simulink model "nmm2d"  (R2025a)
settings: Solver=ode15s  StartTime=0.0  StopTime=20  FixedStep=1e-3  MaxStep=ts_max  RelTol=1e-3  AbsTol=1e-4  EnableMultiTasking=on
values from neighbouring files (symbols this model uses):
  c = 0.05    [nmm2d_mInit.m]
  c_jointstop = 0.3 / (pi/180)    (= 17.1887338539)    [nmm2d_mInit.m]
  D12_F = 0.16    [nmm2d_mInit.m]
  D12_S = L_S    (= 0.5)    [nmm2d_mInit.m]
  D12_T = L_T    (= 0.5)    [nmm2d_mInit.m]
  D1G_F = 0.14    [nmm2d_mInit.m]
  D1G_HAT = 0.35    [nmm2d_mInit.m]
  D1G_S = 0.3    [nmm2d_mInit.m]
  D1G_T = 0.3    [nmm2d_mInit.m]
  DeltaThRef = 5e-3    (= 0.005)    [nmm2d_mInit.m]
  eref = 0.04    [nmm2d_mInit.m]
  FmaxVec = [FmaxSOL FmaxTA FmaxGAS FmaxVAS FmaxHAM FmaxGLU FmaxHFL               FmaxSOL FmaxTA FmaxGAS FmaxVAS FmaxHAM FmaxGLU FmaxHFL]'    [nmm2d_mInit.m]
  g = 9.81    [nmm2d_mInit.m]
  GainDeltaTheta = 2 /100*180/pi    (= 1.14591559026)    [nmm2d_cInit.m]
  GainGAS = 1.1/FmaxGAS    [nmm2d_cInit.m]
  GainGLU = 0.5/FmaxGLU    [nmm2d_cInit.m]
  GainHAM = 0.65/FmaxHAM    [nmm2d_cInit.m]
  GainHAMHFL = 4    [nmm2d_cInit.m]
  GainHFL = 0.5    [nmm2d_cInit.m]
  GainKneOverExt = 2    [nmm2d_cInit.m]
  GainSOL = 1.2/FmaxSOL    [nmm2d_cInit.m]
  GainSOLTA = 0.4/FmaxSOL    [nmm2d_cInit.m]
  GainTA = 1.1    [nmm2d_cInit.m]
  GainVAS = 1.2/FmaxVAS    [nmm2d_cInit.m]
  HAT_CG0 = [-D12_F; 0] + Rot120*[L_S;0] + Rot120*Rot230*[-L_T;0]            + Rot120*Rot230*Rot340*[D1G_HAT;0]    [nmm2d_cInit.m]
  In_F = 0.005    [nmm2d_mInit.m]
  In_HAT = 3    [nmm2d_mInit.m]
  In_S = 0.05    [nmm2d_mInit.m]
  In_T = 0.15    [nmm2d_mInit.m]
  K = 5    [nmm2d_mInit.m]
  k_gx = (2*(m_F+m_S+m_T)+m_HAT)*g/0.1    (= 7848)    [nmm2d_mInit.m]
  k_gy = (2*(m_F+m_S+m_T)+m_HAT)*g/0.01    (= 78480)    [nmm2d_mInit.m]
  k_pressure = m_HAT * 9.81 / DeltaThRef    (= 104967)    [nmm2d_mInit.m]
  K_swing = 0.25    [nmm2d_cInit.m]
  KneePh23Offset = 170*pi/180    (= 2.96705972839)    [nmm2d_cInit.m]
  L_F = 0.2    [nmm2d_mInit.m]
  L_HAT = 0.8    [nmm2d_mInit.m]
  L_S = 0.5    [nmm2d_mInit.m]
  L_T = 0.5    [nmm2d_mInit.m]
  LceOffsetHAM = 0.85    [nmm2d_cInit.m]
  LceOffsetHFL = 0.65    [nmm2d_cInit.m]
  LceOffsetTA = 1-0.5*w    [nmm2d_cInit.m]
  LongDelay = 0.020    (= 0.02)    [nmm2d_cInit.m]
  loptGAS = 0.05    [nmm2d_mInit.m]
  loptGLU = 0.11    [nmm2d_mInit.m]
  loptHAM = 0.10    (= 0.1)    [nmm2d_mInit.m]
  loptHFL = 0.11    [nmm2d_mInit.m]
  loptSOL = 0.04    [nmm2d_mInit.m]
  loptTA = 0.06    [nmm2d_mInit.m]
  loptVAS = 0.08    [nmm2d_mInit.m]
  loptVec = [loptSOL loptTA loptGAS loptVAS loptHAM loptGLU loptHFL               loptSOL loptTA loptGAS loptVAS loptHAM loptGLU loptHFL]'    [nmm2d_mInit.m]
  Lphi120 = 85*pi/180    (= 1.4835298642)    [nmm2d_cInit.m]
  Lphi230 = 175*pi/180    (= 3.05432619099)    [nmm2d_cInit.m]
  Lphi340 = 175*pi/180    (= 3.05432619099)    [nmm2d_cInit.m]
  lslackGAS = 0.40    (= 0.4)    [nmm2d_mInit.m]
  lslackGLU = 0.13    [nmm2d_mInit.m]
  lslackHAM = 0.31    [nmm2d_mInit.m]
  lslackHFL = 0.10    (= 0.1)    [nmm2d_mInit.m]
  lslackSOL = 0.26    [nmm2d_mInit.m]
  lslackTA = 0.24    [nmm2d_mInit.m]
  lslackVAS = 0.23    [nmm2d_mInit.m]
  lslackVec = [lslackSOL lslackTA lslackGAS lslackVAS lslackHAM lslackGLU lslackHFL                 lslackSOL lslackTA lslackGAS lslackVAS lslackHAM lslackGLU lslackHFL]'    [nmm2d_mInit.m]
  m_F = 1.25    [nmm2d_mInit.m]
  m_HAT = 53.5    [nmm2d_mInit.m]
  m_S = 3.5    [nmm2d_mInit.m]
  m_T = 8.5    [nmm2d_mInit.m]
  MidDelay = 0.010    (= 0.01)    [nmm2d_cInit.m]
  mu_slide = 0.8    [nmm2d_mInit.m]
  mu_stick = 0.9    [nmm2d_mInit.m]
  N = 1.5    [nmm2d_mInit.m]
  phi12_LowLimit = 70*pi/180    (= 1.2217304764)    [nmm2d_mInit.m]
  phi12_UpLimit = 130*pi/180    (= 2.26892802759)    [nmm2d_mInit.m]
  phi23_UpLimit = 175*pi/180    (= 3.05432619099)    [nmm2d_mInit.m]
  phi34_UpLimit = 230*pi/180    (= 4.01425727959)    [nmm2d_mInit.m]
  phimaxGASa = 110*pi/180    (= 1.91986217719)    [nmm2d_mInit.m]
  phimaxGASk = 140*pi/180    (= 2.44346095279)    [nmm2d_mInit.m]
  phimaxHAMk = 180*pi/180    (= 3.14159265359)    [nmm2d_mInit.m]
  phimaxSOL = 110*pi/180    (= 1.91986217719)    [nmm2d_mInit.m]
  phimaxTA = 80*pi/180    (= 1.3962634016)    [nmm2d_mInit.m]
  phimaxVAS = 165*pi/180    (= 2.87979326579)    [nmm2d_mInit.m]
  phirefGASa = 80*pi/180    (= 1.3962634016)    [nmm2d_mInit.m]
  phirefGASk = 165*pi/180    (= 2.87979326579)    [nmm2d_mInit.m]
  phirefGLU = 150*pi/180    (= 2.61799387799)    [nmm2d_mInit.m]
  phirefHAMh = 155*pi/180    (= 2.70526034059)    [nmm2d_mInit.m]
  phirefHAMk = 180*pi/180    (= 3.14159265359)    [nmm2d_mInit.m]
  phirefHFL = 180*pi/180    (= 3.14159265359)    [nmm2d_mInit.m]
  phirefSOL = 80*pi/180    (= 1.3962634016)    [nmm2d_mInit.m]
  phirefTA = 110*pi/180    (= 1.91986217719)    [nmm2d_mInit.m]
  phirefVAS = 125*pi/180    (= 2.18166156499)    [nmm2d_mInit.m]
  PosGainGG = 1/(30*pi/180)    (= 1.9098593171)    [nmm2d_cInit.m]
  preA = 0.01    [nmm2d_mInit.m]
  PreStimGAS = 0.01    [nmm2d_cInit.m]
  PreStimGG = 0.05    [nmm2d_cInit.m]
  PreStimGLU = 0.01    [nmm2d_cInit.m]
  PreStimHAM = 0.01    [nmm2d_cInit.m]
  PreStimHFL = 0.01    [nmm2d_cInit.m]
  PreStimSOL = 0.01    [nmm2d_cInit.m]
  PreStimTA = 0.01    [nmm2d_cInit.m]
  PreStimVAS = 0.08    [nmm2d_cInit.m]
  rGASa = 0.05    [nmm2d_mInit.m]
  rGASk = 0.05    [nmm2d_mInit.m]
  rGLU = 0.10    (= 0.1)    [nmm2d_mInit.m]
  rHAMh = 0.08    [nmm2d_mInit.m]
  rHAMk = 0.05    [nmm2d_mInit.m]
  rHFL = 0.10    (= 0.1)    [nmm2d_mInit.m]
  rhoGASa = 0.7    [nmm2d_mInit.m]
  rhoGASk = 0.7    [nmm2d_mInit.m]
  rhoGLU = 0.5    [nmm2d_mInit.m]
  rhoHAMh = 0.7    [nmm2d_mInit.m]
  rhoHAMk = 0.7    [nmm2d_mInit.m]
  rhoHFL = 0.5    [nmm2d_mInit.m]
  rhoSOL = 0.5    [nmm2d_mInit.m]
  rhoTA = 0.7    [nmm2d_mInit.m]
  rhoVAS = 0.7    [nmm2d_mInit.m]
  Rphi120 = 90*pi/180    (= 1.57079632679)    [nmm2d_cInit.m]
  Rphi230 = 175*pi/180    (= 3.05432619099)    [nmm2d_cInit.m]
  Rphi340 = 140*pi/180    (= 2.44346095279)    [nmm2d_cInit.m]
  rSOL = 0.05    [nmm2d_mInit.m]
  rTA = 0.04    [nmm2d_mInit.m]
  rVAS = 0.06    [nmm2d_mInit.m]
  ... (+12 more)
undefined symbols (not defined in the file or in its folder): sgn, X, Y, Z
libraries: sm_lib x70, nesl_utility x67, simulink x27, simulink_extras x6
(part 1 of 5)
settings Model: Creator=hgeyer  LastModifiedBy=hgeyer
settings SolverCC: AutoScaleAbsTol=off  AlgebraicLoopSolver=TrustRegion
settings DataIOCC: SaveFormat=Array  SignalLoggingSaveFormat=ModelDataLogs  SignalLogging=off  ReturnWorkspaceOutputs=off
settings OptimizationCC: BooleanDataType=off  ExpressionDepthLimit=2147483647.0  InitFltsAndDblsToZero=on  LifeSpan=inf
settings DebuggingCC: SaveWithParameterizedLinksMsg=none  UnderspecifiedInitializationDetection=Classic  MergeDetectMultiDrivingBlocksExec=none  SignalResolutionControl=TryResolveAllWithWarning  SolverPrmCheckMsg=warning  MultiTaskDSMMsg=warning  MultiTaskCondExecSysMsg=none  FcnCallInpInsideContextMsg=warning  UnconnectedInputMsg=warning  UnconnectedOutputMsg=warning  UnconnectedLineMsg=warning  StateNameClashWarn=warning  SFUnexpectedBacktrackingDiag=warning  SFNoUnconditionalDefaultTransitionDiag=warning  SFExecutionAtInitializationDiag=none  ArithmeticOperatorsInVariantConditions=warning
settings HardwareCC: ProdBitPerPointer=32.0  ProdBitPerSizeT=32.0  ProdBitPerPtrDiffT=32.0  ProdLargestAtomicFloat=None  ProdIntDivRoundTo=Undefined  ProdEndianess=Unspecified  ProdWordSize=32.0  ProdHWDeviceType=32-bit Generic
settings ModelReferenceCC: EnableRefExpFcnMdlSchedulingChecks=on  PropagateSignalLabelsOutOfModel=off
settings SFSimCC: SimUseLocalCustomCode=off  CustomCodeUndefinedFunction=UseInterfaceOnly
settings RTWCC: RTWUseLocalCustomCode=off  GPUComputeCapability=3.5  DLArmComputeVersion=19.05
settings CodeAppCC: StateflowObjectComments=on
settings GRTTargetCC: TargetFcnLib=ansi_tfl_tmw.mat  TargetLangStandard=C89/C90 (ANSI)  CombineOutputUpdateFcns=off  GRTInterface=on
settings ConfigComp: CovMetricSettings=dw  CovSaveCumulativeToWorkspaceVar=on  CovSaveSingleToWorkspaceVar=on  CovExternalEMLEnable=off
settings SimscapeCC: SimscapeNormalizeSystem=off
settings ConfigurationSet: Description=SimMechanics 2G
settings ExplorerConfigSet: InternalSimMechanicsExplorerSettings="<ExplorerConfiguration><canonicalview>planar_xy</canonicalview><TilePanel><TileInfo><Tiles Columns=\"1\" Count=\"1\" Height=\"642\" Rows=\"1\" Width=\"1726\"><Row Weight=\"1\"/><Column Weight=\"1\"/><Tile Height=\"1\" Width=\"1\" X=\"0\" Y=\"0\"/></Tiles></TileInfo><SceneInfo><SceneViewer><IsThisViewStd><IsStandardView>off</IsStandardView><StandardViewName>Front</StandardViewName></IsThisViewStd><BGColor><R>0.80000000000000004</R><G>0.80000000000000004</G><B>0.80000000000000004</B><A>1</A></BGColor><Camera><DoPerspective>off</DoPerspective><Position><X>4.801317548788429</X><Y>1.5671458374770342</Y><Z>5.9284706387938888</Z></Position><Center><X>4.801317548788429</X><Y>1.5671458374770342</Y><Z>-1.0408340855860843e-17</Z></Center><Up><X>0</X><Y>1</Y><Z>0</Z></Up><XLim>1.9471871489356678</XLim><YLim>1.9471871489356678</YLim><ViewLimDist>0.01</ViewLimDist></Camera></SceneViewer></SceneInfo></TilePanel><MechEditorPanel><GfxPanelCameraMap/><Cameras/><VideoCreator><IncludeTiles>All</IncludeTiles><IncludeTime>on</IncludeTime><IncludeWorldFrame>off</IncludeWorldFrame><PlaybackSpeedRatio>1</PlaybackSpeedRatio><FrameRate>30</FrameRate><FrameSize>auto</FrameSize><VideoFormat>MPEG4</VideoFormat></VideoCreator></MechEditorPanel><PlaybackSettings><PlaybackSpeedFactor>1</PlaybackSpeedFactor></PlaybackSettings></ExplorerConfiguration>"

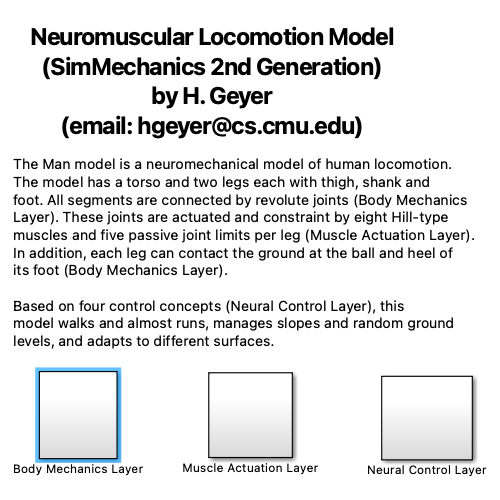
[thumbnail: Simulink's stored preview of the top-level diagram]
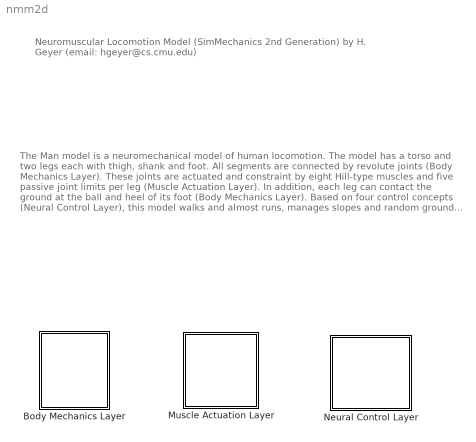
== system nmm2d ==
  note: The Man model is a neuromechanical model of human locomotion.
      | The model has a torso and two legs each with thigh, shank and
      | foot. All segments are connected by revolute joints (Body Mechanics
      | Layer). These joints are actuated and constraint by eight Hill-type
      | muscles and five passive joint limits per leg (Muscle Actuation Layer).
      | In addition, each leg can contact the ground at the ball and heel of
      | its foot (Body Mechanics Layer).
      |
      | Based on four control concepts (Neural Control Layer), this
      | model walks and almost runs, manages slopes and random ground
      | levels, and adapts to different surfaces.
  note: Neuromuscular Locomotion Model
      | (SimMechanics 2nd Generation)
      | by H. Geyer
      | (email: hgeyer@cs.cmu.edu)
  Body Mechanics Layer : Subsystem
  Muscle Actuation Layer : Subsystem
  Neural Control Layer : Subsystem

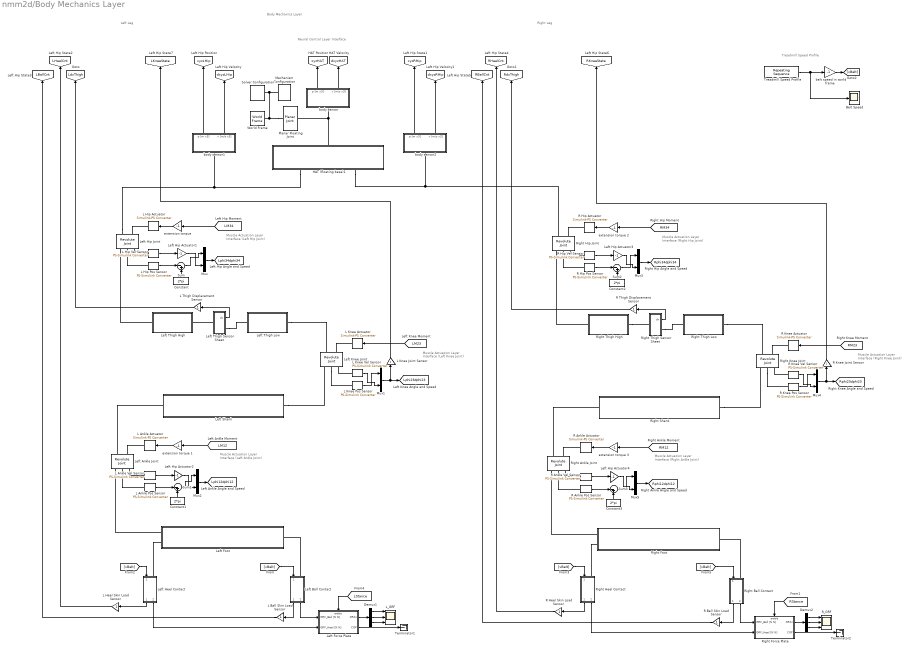
== system nmm2d/Body Mechanics Layer ==
  note: Treadmill Speed Profile
  note: Left Leg
  note: Body Mechanics Layer
  note: Neural Control Layer Interface
  note: Muscle Actuation
      | Layer Interface
      | (Left Hip Joint)
  note: Muscle Actuation
      | Layer Interface
      | (Right Ankle Joint)
  note: Muscle Actuation
      | Layer Interface
      | (Left Knee Joint)
  note: Right Leg
  note: Muscle Actuation
      | Layer Interface
      | (Right Knee Joint)
  note: Muscle Actuation
      | Layer Interface
      | (Left Ankle Joint)
  note: Muscle Actuation
      | Layer Interface
      | (Right Hip Joint)
  Belt Speed : Scope
      settings: TimeSpan=3  ActiveDisplayYMinimum=-0.14999999999999997  ActiveDisplayYMaximum=1.3499999999999999  DataLoggingSaveFormat=Array
  Constant{,1..3} (4 alike) : Constant  Value=2*pi
  Demux1 : Demux  Outputs=3
  Demux2 : Demux  Outputs=3
  HAT (floating base)1 : Subsystem
  L Ankle Actuator : nesl_utility/Simulink-PS Converter  PhysicalDomain=network_engine_domain  SubClassName=ps_input  LeftPortType=input  RightPortType=output  PseudoPeriodic=off  Frequencies=[]  NoiseDistribution=none  NoiseParameters=[]  Unit=N*m  AffineConversion=off  FilteringAndDerivatives=zero  SimscapeFilterOrder=1  InputFilterTimeConstant=.001  UdotUserProvided=0
  L Ankle Vel Sensor : nesl_utility/PS-Simulink Converter  PhysicalDomain=network_engine_domain  SubClassName=ps_output  LeftPortType=input  RightPortType=output  PseudoPeriodic=off  Frequencies=[]  VectorFormat=1-D array  Unit=rad/s  AffineConversion=off
  L Ankle Pos Sensor : nesl_utility/PS-Simulink Converter  PhysicalDomain=network_engine_domain  SubClassName=ps_output  LeftPortType=input  RightPortType=output  PseudoPeriodic=off  Frequencies=[]  VectorFormat=1-D array  Unit=rad  AffineConversion=off
  L Ball Skin Load Sensor : Gain
  L Heel Skin Load Sensor : Gain
  L Hip Actuator : nesl_utility/Simulink-PS Converter  PhysicalDomain=network_engine_domain  SubClassName=ps_input  LeftPortType=input  RightPortType=output  PseudoPeriodic=off  Frequencies=[]  NoiseDistribution=none  NoiseParameters=[]  Unit=N*m  AffineConversion=off  FilteringAndDerivatives=zero  SimscapeFilterOrder=1  InputFilterTimeConstant=.001  UdotUserProvided=0
  L Hip Vel Sensor : nesl_utility/PS-Simulink Converter  PhysicalDomain=network_engine_domain  SubClassName=ps_output  LeftPortType=input  RightPortType=output  PseudoPeriodic=off  Frequencies=[]  VectorFormat=1-D array  Unit=rad/s  AffineConversion=off
  L Hip Pos Sensor : nesl_utility/PS-Simulink Converter  PhysicalDomain=network_engine_domain  SubClassName=ps_output  LeftPortType=input  RightPortType=output  PseudoPeriodic=off  Frequencies=[]  VectorFormat=1-D array  Unit=rad  AffineConversion=off
  L Knee Actuator : nesl_utility/Simulink-PS Converter  PhysicalDomain=network_engine_domain  SubClassName=ps_input  LeftPortType=input  RightPortType=output  PseudoPeriodic=off  Frequencies=[]  NoiseDistribution=none  NoiseParameters=[]  Unit=N*m  AffineConversion=off  FilteringAndDerivatives=zero  SimscapeFilterOrder=1  InputFilterTimeConstant=.001  UdotUserProvided=0
  L Knee Joint Sensor : Gain
  L Knee Vel Sensor : nesl_utility/PS-Simulink Converter  PhysicalDomain=network_engine_domain  SubClassName=ps_output  LeftPortType=input  RightPortType=output  PseudoPeriodic=off  Frequencies=[]  VectorFormat=1-D array  Unit=rad/s  AffineConversion=off
  L Knee Pos Sensor : nesl_utility/PS-Simulink Converter  PhysicalDomain=network_engine_domain  SubClassName=ps_output  LeftPortType=input  RightPortType=output  PseudoPeriodic=off  Frequencies=[]  VectorFormat=1-D array  Unit=rad  AffineConversion=off
  L Thigh Displacement  Sensor : Gain
  L_GRF : Scope  NumInputPorts=3
      settings: TimeSpan=3  ActiveDisplayYMinimum=-1040.11321  ActiveDisplayYMaximum=4604.02049  DataLoggingSaveFormat=Array
  Left Ankle Joint : sm_lib/Joints/Revolute Joint  JointMode=Normal  CompositeWrenchDir=FollowerOnBase  CompositeWrenchFrame=BaseFrame  SenseConstraintForce=off  SenseConstraintTorque=off  SenseTotalForce=off  SenseTotalTorque=off  PositionTargetSpecify=on  PositionTargetPriority=High  PositionTargetValue=2*pi-Lphi120  PositionTargetValueUnits=rad  VelocityTargetSpecify=on  VelocityTargetPriority=High  VelocityTargetValue=0  VelocityTargetValueUnits=rad/s  EquilibriumPosition=0  EquilibriumPositionUnits=deg  SpringStiffness=0  SpringStiffnessUnits=N*m/deg  DampingCoefficient=0  DampingCoefficientUnits=N*m/(deg/s)  LowerLimitSpecify=off  LowerLimitBound=-90  LowerLimitBoundUnits=deg  LowerLimitStiffness=1e4  LowerLimitStiffnessUnits=N*m/deg  LowerLimitDamping=10  LowerLimitDampingUnits=N*m/(deg/s)  LowerLimitTransitionRegionWidth=0.1  LowerLimitTransitionRegionWidthUnits=deg  UpperLimitSpecify=off  UpperLimitBound=90  UpperLimitBoundUnits=deg  UpperLimitStiffness=1e4  UpperLimitStiffnessUnits=N*m/deg  UpperLimitDamping=10  UpperLimitDampingUnits=N*m/(deg/s)  UpperLimitTransitionRegionWidth=0.1  UpperLimitTransitionRegionWidthUnits=deg  TorqueActuationMode=InputTorque  MotionActuationMode=ComputedMotion  SensePosition=on  SenseVelocity=on  SenseAcceleration=off  SenseTorqueForce=off  SenseLowerLimitTorqueForce=off  SenseUpperLimitTorqueForce=off
  Left Ball Contact : Subsystem
  Left Heel Contact : Subsystem
  Left Hip Joint : sm_lib/Joints/Revolute Joint  JointMode=Normal  CompositeWrenchDir=FollowerOnBase  CompositeWrenchFrame=BaseFrame  SenseConstraintForce=off  SenseConstraintTorque=off  SenseTotalForce=off  SenseTotalTorque=off  PositionTargetSpecify=on  PositionTargetPriority=High  PositionTargetValue=2*pi-Lphi340  PositionTargetValueUnits=rad  VelocityTargetSpecify=on  VelocityTargetPriority=High  VelocityTargetValue=0  VelocityTargetValueUnits=rad/s  EquilibriumPosition=0  EquilibriumPositionUnits=deg  SpringStiffness=0  SpringStiffnessUnits=N*m/deg  DampingCoefficient=0  DampingCoefficientUnits=N*m/(deg/s)  LowerLimitSpecify=off  LowerLimitBound=-90  LowerLimitBoundUnits=deg  LowerLimitStiffness=1e4  LowerLimitStiffnessUnits=N*m/deg  LowerLimitDamping=10  LowerLimitDampingUnits=N*m/(deg/s)  LowerLimitTransitionRegionWidth=0.1  LowerLimitTransitionRegionWidthUnits=deg  UpperLimitSpecify=off  UpperLimitBound=90  UpperLimitBoundUnits=deg  UpperLimitStiffness=1e4  UpperLimitStiffnessUnits=N*m/deg  UpperLimitDamping=10  UpperLimitDampingUnits=N*m/(deg/s)  UpperLimitTransitionRegionWidth=0.1  UpperLimitTransitionRegionWidthUnits=deg  TorqueActuationMode=InputTorque  MotionActuationMode=ComputedMotion  SensePosition=on  SenseVelocity=on  SenseAcceleration=off  SenseTorqueForce=off  SenseLowerLimitTorqueForce=off  SenseUpperLimitTorqueForce=off
  Left Knee Joint : sm_lib/Joints/Revolute Joint  JointMode=Normal  CompositeWrenchDir=FollowerOnBase  CompositeWrenchFrame=BaseFrame  SenseConstraintForce=off  SenseConstraintTorque=off  SenseTotalForce=off  SenseTotalTorque=off  PositionTargetSpecify=on  PositionTargetPriority=High  PositionTargetValue=Lphi230  PositionTargetValueUnits=rad  VelocityTargetSpecify=on  VelocityTargetPriority=High  VelocityTargetValue=0  VelocityTargetValueUnits=rad/s  EquilibriumPosition=0  EquilibriumPositionUnits=deg  SpringStiffness=0  SpringStiffnessUnits=N*m/deg  DampingCoefficient=0  DampingCoefficientUnits=N*m/(deg/s)  LowerLimitSpecify=off  LowerLimitBound=-90  LowerLimitBoundUnits=deg  LowerLimitStiffness=1e4  LowerLimitStiffnessUnits=N*m/deg  LowerLimitDamping=10  LowerLimitDampingUnits=N*m/(deg/s)  LowerLimitTransitionRegionWidth=0.1  LowerLimitTransitionRegionWidthUnits=deg  UpperLimitSpecify=off  UpperLimitBound=90  UpperLimitBoundUnits=deg  UpperLimitStiffness=1e4  UpperLimitStiffnessUnits=N*m/deg  UpperLimitDamping=10  UpperLimitDampingUnits=N*m/(deg/s)  UpperLimitTransitionRegionWidth=0.1  UpperLimitTransitionRegionWidthUnits=deg  TorqueActuationMode=InputTorque  MotionActuationMode=ComputedMotion  SensePosition=on  SenseVelocity=on  SenseAcceleration=off  SenseTorqueForce=off  SenseLowerLimitTorqueForce=off  SenseUpperLimitTorqueForce=off
  Left Foot : Subsystem
  Left Force Plate : Subsystem  TreatAsAtomicUnit=on
  Left Hip Actuator{1..4} (4 alike) : Gain  Gain=-1
  "Left Shank " : Subsystem
  Left Thigh Sensor Sheet : Subsystem
  Left Thigh High : Subsystem
  Left Thigh Low : Subsystem
  Mechanism Configuration : sm_lib/Utilities/Mechanism Configuration  UniformGravity=Constant  GravityVector=[0 -9.81 0]  GravityVectorUnits=m/s^2  LinearizationDelta=0.001  JointModeTransitionNonlinearIterations=2
  Mux{,1..5} (6 alike) : Mux  Inputs=2
  "Planar Floating Joint " : sm_lib/Joints/Planar Joint  JointMode=Normal  CompositeWrenchDir=FollowerOnBase  CompositeWrenchFrame=BaseFrame  SenseConstraintForce=off  SenseConstraintTorque=off  SenseTotalForce=off  SenseTotalTorque=off  PxPositionTargetSpecify=on  PxPositionTargetPriority=High  PxPositionTargetValue=HAT_CG0(1)  PxPositionTargetValueUnits=m  PxVelocityTargetSpecify=on  PxVelocityTargetPriority=High  PxVelocityTargetValue=vx0  PxVelocityTargetValueUnits=m/s  PxEquilibriumPosition=0  PxEquilibriumPositionUnits=m  PxSpringStiffness=0  PxSpringStiffnessUnits=N/m  PxDampingCoefficient=0  PxDampingCoefficientUnits=N/(m/s)  PxLowerLimitSpecify=off  PxLowerLimitBound=-1  PxLowerLimitBoundUnits=m  PxLowerLimitStiffness=1e6  PxLowerLimitStiffnessUnits=N/m  PxLowerLimitDamping=1e3  PxLowerLimitDampingUnits=N/(m/s)  PxLowerLimitTransitionRegionWidth=1e-4  PxLowerLimitTransitionRegionWidthUnits=m  PxUpperLimitSpecify=off  PxUpperLimitBound=1  PxUpperLimitBoundUnits=m  PxUpperLimitStiffness=1e6  PxUpperLimitStiffnessUnits=N/m  PxUpperLimitDamping=1e3  PxUpperLimitDampingUnits=N/(m/s)  PxUpperLimitTransitionRegionWidth=1e-4  PxUpperLimitTransitionRegionWidthUnits=m  PxTorqueActuationMode=NoTorque  PxMotionActuationMode=ComputedMotion  PxSensePosition=off  PxSenseVelocity=off  PxSenseAcceleration=off  PxSenseTorqueForce=off  PxSenseLowerLimitTorqueForce=off  PxSenseUpperLimitTorqueForce=off  PyPositionTargetSpecify=on  PyPositionTargetPriority=High  PyPositionTargetValue=HAT_CG0(2)  PyPositionTargetValueUnits=m  PyVelocityTargetSpecify=on  PyVelocityTargetPriority=High  PyVelocityTargetValue=0  PyVelocityTargetValueUnits=m/s  PyEquilibriumPosition=0  PyEquilibriumPositionUnits=m  PySpringStiffness=0  PySpringStiffnessUnits=N/m  PyDampingCoefficient=0  PyDampingCoefficientUnits=N/(m/s)  PyLowerLimitSpecify=off  PyLowerLimitBound=-1  PyLowerLimitBoundUnits=m  PyLowerLimitStiffness=1e6  PyLowerLimitStiffnessUnits=N/m  PyLowerLimitDamping=1e3  PyLowerLimitDampingUnits=N/(m/s)  PyLowerLimitTransitionRegionWidth=1e-4  PyLowerLimitTransitionRegionWidthUnits=m  PyUpperLimitSpecify=off  PyUpperLimitBound=1  PyUpperLimitBoundUnits=m  PyUpperLimitStiffness=1e6  PyUpperLimitStiffnessUnits=N/m  PyUpperLimitDamping=1e3  PyUpperLimitDampingUnits=N/(m/s)  PyUpperLimitTransitionRegionWidth=1e-4  PyUpperLimitTransitionRegionWidthUnits=m  PyTorqueActuationMode=NoTorque  PyMotionActuationMode=ComputedMotion  PySensePosition=off  PySenseVelocity=off  PySenseAcceleration=off  PySenseTorqueForce=off  PySenseLowerLimitTorqueForce=off  PySenseUpperLimitTorqueForce=off  RzPositionTargetSpecify=on  RzPositionTargetPriority=High  RzPositionTargetValue=(Lphi120-Lphi230+Lphi340)-pi/2  RzPositionTargetValueUnits=rad  RzVelocityTargetSpecify=on  RzVelocityTargetPriority=High  RzVelocityTargetValue=0  RzVelocityTargetValueUnits=deg/s  RzEquilibriumPosition=0  RzEquilibriumPositionUnits=deg  RzSpringStiffness=0  RzSpringStiffnessUnits=N*m/deg  RzDampingCoefficient=0  RzDampingCoefficientUnits=N*m/(deg/s)  RzLowerLimitSpecify=off  RzLowerLimitBound=-90  RzLowerLimitBoundUnits=deg  RzLowerLimitStiffness=1e4  RzLowerLimitStiffnessUnits=N*m/deg  RzLowerLimitDamping=10  RzLowerLimitDampingUnits=N*m/(deg/s)  RzLowerLimitTransitionRegionWidth=0.1  RzLowerLimitTransitionRegionWidthUnits=deg  RzUpperLimitSpecify=off  RzUpperLimitBound=90  RzUpperLimitBoundUnits=deg  RzUpperLimitStiffness=1e4  RzUpperLimitStiffnessUnits=N*m/deg  RzUpperLimitDamping=10  RzUpperLimitDampingUnits=N*m/(deg/s)  RzUpperLimitTransitionRegionWidth=0.1  RzUpperLimitTransitionRegionWidthUnits=deg  RzTorqueActuationMode=NoTorque  RzMotionActuationMode=ComputedMotion  RzSensePosition=off  RzSenseVelocity=off  RzSenseAcceleration=off  RzSenseTorqueForce=off  RzSenseLowerLimitTorqueForce=off  RzSenseUpperLimitTorqueForce=off
  R Ankle Actuator : nesl_utility/Simulink-PS Converter  PhysicalDomain=network_engine_domain  SubClassName=ps_input  LeftPortType=input  RightPortType=output  PseudoPeriodic=off  Frequencies=[]  NoiseDistribution=none  NoiseParameters=[]  Unit=N*m  AffineConversion=off  FilteringAndDerivatives=zero  SimscapeFilterOrder=1  InputFilterTimeConstant=.001  UdotUserProvided=0
  R Ankle Vel Sensor : nesl_utility/PS-Simulink Converter  PhysicalDomain=network_engine_domain  SubClassName=ps_output  LeftPortType=input  RightPortType=output  PseudoPeriodic=off  Frequencies=[]  VectorFormat=1-D array  Unit=rad/s  AffineConversion=off
  R Ankle Pos Sensor : nesl_utility/PS-Simulink Converter  PhysicalDomain=network_engine_domain  SubClassName=ps_output  LeftPortType=input  RightPortType=output  PseudoPeriodic=off  Frequencies=[]  VectorFormat=1-D array  Unit=rad  AffineConversion=off
  R Ball Skin Load Sensor : Gain
  R Heel Skin Load Sensor : Gain
  R Hip Actuator : nesl_utility/Simulink-PS Converter  PhysicalDomain=network_engine_domain  SubClassName=ps_input  LeftPortType=input  RightPortType=output  PseudoPeriodic=off  Frequencies=[]  NoiseDistribution=none  NoiseParameters=[]  Unit=N*m  AffineConversion=off  FilteringAndDerivatives=zero  SimscapeFilterOrder=1  InputFilterTimeConstant=.001  UdotUserProvided=0
  R Hip Vel Sensor : nesl_utility/PS-Simulink Converter  PhysicalDomain=network_engine_domain  SubClassName=ps_output  LeftPortType=input  RightPortType=output  PseudoPeriodic=off  Frequencies=[]  VectorFormat=1-D array  Unit=rad/s  AffineConversion=off
  R Hip Pos Sensor : nesl_utility/PS-Simulink Converter  PhysicalDomain=network_engine_domain  SubClassName=ps_output  LeftPortType=input  RightPortType=output  PseudoPeriodic=off  Frequencies=[]  VectorFormat=1-D array  Unit=rad  AffineConversion=off
  R Knee Actuator : nesl_utility/Simulink-PS Converter  PhysicalDomain=network_engine_domain  SubClassName=ps_input  LeftPortType=input  RightPortType=output  PseudoPeriodic=off  Frequencies=[]  NoiseDistribution=none  NoiseParameters=[]  Unit=N*m  AffineConversion=off  FilteringAndDerivatives=zero  SimscapeFilterOrder=1  InputFilterTimeConstant=.001  UdotUserProvided=0
  R Knee Joint Sensor : Gain
  R Knee Vel Sensor : nesl_utility/PS-Simulink Converter  PhysicalDomain=network_engine_domain  SubClassName=ps_output  LeftPortType=input  RightPortType=output  PseudoPeriodic=off  Frequencies=[]  VectorFormat=1-D array  Unit=rad/s  AffineConversion=off
  R Knee Pos Sensor : nesl_utility/PS-Simulink Converter  PhysicalDomain=network_engine_domain  SubClassName=ps_output  LeftPortType=input  RightPortType=output  PseudoPeriodic=off  Frequencies=[]  VectorFormat=1-D array  Unit=rad  AffineConversion=off
  R Thigh Displacement  Sensor : Gain
  R_GRF : Scope  NumInputPorts=3
      settings: TimeSpan=3  ActiveDisplayYMinimum=-2014.79592  ActiveDisplayYMaximum=3935.07816  DataLoggingSaveFormat=Array
  Right Ankle Joint : sm_lib/Joints/Revolute Joint  JointMode=Normal  CompositeWrenchDir=FollowerOnBase  CompositeWrenchFrame=BaseFrame  SenseConstraintForce=off  SenseConstraintTorque=off  SenseTotalForce=off  SenseTotalTorque=off  PositionTargetSpecify=on  PositionTargetPriority=High  PositionTargetValue=2*pi-Rphi120  PositionTargetValueUnits=rad  VelocityTargetSpecify=on  VelocityTargetPriority=High  VelocityTargetValue=0  VelocityTargetValueUnits=rad/s  EquilibriumPosition=0  EquilibriumPositionUnits=deg  SpringStiffness=0  SpringStiffnessUnits=N*m/deg  DampingCoefficient=0  DampingCoefficientUnits=N*m/(deg/s)  LowerLimitSpecify=off  LowerLimitBound=-90  LowerLimitBoundUnits=deg  LowerLimitStiffness=1e4  LowerLimitStiffnessUnits=N*m/deg  LowerLimitDamping=10  LowerLimitDampingUnits=N*m/(deg/s)  LowerLimitTransitionRegionWidth=0.1  LowerLimitTransitionRegionWidthUnits=deg  UpperLimitSpecify=off  UpperLimitBound=90  UpperLimitBoundUnits=deg  UpperLimitStiffness=1e4  UpperLimitStiffnessUnits=N*m/deg  UpperLimitDamping=10  UpperLimitDampingUnits=N*m/(deg/s)  UpperLimitTransitionRegionWidth=0.1  UpperLimitTransitionRegionWidthUnits=deg  TorqueActuationMode=InputTorque  MotionActuationMode=ComputedMotion  SensePosition=on  SenseVelocity=on  SenseAcceleration=off  SenseTorqueForce=off  SenseLowerLimitTorqueForce=off  SenseUpperLimitTorqueForce=off
  Right Ball Contact : Subsystem
  Right Heel Contact : Subsystem
  Right Hip Joint : sm_lib/Joints/Revolute Joint  JointMode=Normal  CompositeWrenchDir=FollowerOnBase  CompositeWrenchFrame=BaseFrame  SenseConstraintForce=off  SenseConstraintTorque=off  SenseTotalForce=off  SenseTotalTorque=off  PositionTargetSpecify=on  PositionTargetPriority=High  PositionTargetValue=2*pi-Rphi340  PositionTargetValueUnits=rad  VelocityTargetSpecify=on  VelocityTargetPriority=High  VelocityTargetValue=0  VelocityTargetValueUnits=rad/s  EquilibriumPosition=0  EquilibriumPositionUnits=deg  SpringStiffness=0  SpringStiffnessUnits=N*m/deg  DampingCoefficient=0  DampingCoefficientUnits=N*m/(deg/s)  LowerLimitSpecify=off  LowerLimitBound=-90  LowerLimitBoundUnits=deg  LowerLimitStiffness=1e4  LowerLimitStiffnessUnits=N*m/deg  LowerLimitDamping=10  LowerLimitDampingUnits=N*m/(deg/s)  LowerLimitTransitionRegionWidth=0.1  LowerLimitTransitionRegionWidthUnits=deg  UpperLimitSpecify=off  UpperLimitBound=90  UpperLimitBoundUnits=deg  UpperLimitStiffness=1e4  UpperLimitStiffnessUnits=N*m/deg  UpperLimitDamping=10  UpperLimitDampingUnits=N*m/(deg/s)  UpperLimitTransitionRegionWidth=0.1  UpperLimitTransitionRegionWidthUnits=deg  TorqueActuationMode=InputTorque  MotionActuationMode=ComputedMotion  SensePosition=on  SenseVelocity=on  SenseAcceleration=off  SenseTorqueForce=off  SenseLowerLimitTorqueForce=off  SenseUpperLimitTorqueForce=off
  Right Knee Joint : sm_lib/Joints/Revolute Joint  JointMode=Normal  CompositeWrenchDir=FollowerOnBase  CompositeWrenchFrame=BaseFrame  SenseConstraintForce=off  SenseConstraintTorque=off  SenseTotalForce=off  SenseTotalTorque=off  PositionTargetSpecify=on  PositionTargetPriority=High  PositionTargetValue=Rphi230  PositionTargetValueUnits=rad  VelocityTargetSpecify=on  VelocityTargetPriority=High  VelocityTargetValue=0  VelocityTargetValueUnits=rad/s  EquilibriumPosition=0  EquilibriumPositionUnits=deg  SpringStiffness=0  SpringStiffnessUnits=N*m/deg  DampingCoefficient=0  DampingCoefficientUnits=N*m/(deg/s)  LowerLimitSpecify=off  LowerLimitBound=-90  LowerLimitBoundUnits=deg  LowerLimitStiffness=1e4  LowerLimitStiffnessUnits=N*m/deg  LowerLimitDamping=10  LowerLimitDampingUnits=N*m/(deg/s)  LowerLimitTransitionRegionWidth=0.1  LowerLimitTransitionRegionWidthUnits=deg  UpperLimitSpecify=off  UpperLimitBound=90  UpperLimitBoundUnits=deg  UpperLimitStiffness=1e4  UpperLimitStiffnessUnits=N*m/deg  UpperLimitDamping=10  UpperLimitDampingUnits=N*m/(deg/s)  UpperLimitTransitionRegionWidth=0.1  UpperLimitTransitionRegionWidthUnits=deg  TorqueActuationMode=InputTorque  MotionActuationMode=ComputedMotion  SensePosition=on  SenseVelocity=on  SenseAcceleration=off  SenseTorqueForce=off  SenseLowerLimitTorqueForce=off  SenseUpperLimitTorqueForce=off
  Right Foot : Subsystem
  Right Force Plate : Subsystem  TreatAsAtomicUnit=on
  Right Shank : Subsystem
  Right Thigh Sensor Sheet : Subsystem
  Right Thigh High : Subsystem
  Right Thigh Low : Subsystem
  Solver Configuration : nesl_utility/Solver Configuration  PhysicalDomain=network_engine_domain  SubClassName=solver  LeftPortType=input  RightPortType=generic  Tones=[]  Harmonics=[]  SimulateNoise=off  Profile=off  UseLocalSampling=off  EnableSwitchedLinearOptims=on  FrequencyDomain=off  UseCCode=off  RelTol=0.001  AbsTol=1e-06  MinStep=1e-09  ToWorkspace=off  RevertToSquareIcSolve=off  NumHomotopyIterations=100  PhasorMode=off  PhasorModeNumHarmonics=1  ConsistencySolver=NEWTON_FTOL  IndexReductionMethod=DerivativeReplacement  DoDC=off  ResidualTolerance=1e-9  ConsistencyTolSource=GLOBAL  ConsistencyAbsTol=0.001  ConsistencyRelTol=0.001  ConsistencyTolFactor=0.001  UseLocalSolver=off  LocalSolverChoice=NE_BACKWARD_EULER_ADVANCER  ResolveIndetEquations=on  FunctionEvalNumThread=1  LocalSolverSampleTime=.001  DoFixedCost=off  MaxNonlinIter=3  MaxModeIter=2  ComputeImpulses=off  ImpulseIterations=2  LinearAlgebra=Sparse  LinearAlgebraNumThread=0  EquationFormulation=NE_TIME_EF  DelaysMemoryBudget=1024  AutomaticFiltering=on  FilteringTimeConstant=0.001  PartitionStorageMethod=AS_NEEDED  PartitionMemoryBudget=1024  PartitionMethod=FAST  MultibodyUseLocalSolver=off  MultibodyLocalSolverChoice=ODE1  MultibodyLocalSolverSampleTime=0.001
  Sum{,1..3} (4 alike) : Sum  Inputs=|-+
  Terminator1 : Terminator
  Terminator2 : Terminator
  Treadmill Speed Profile : simulink/Sources/Repeating Sequence  rep_seq_t=[0 3 8 13 18 20]  rep_seq_y=[0 0 1.2 1.2 0 0]
  World Frame : sm_lib/Frames and Transforms/World Frame
  belt speed in world frame : Gain  Gain=-1
  body sensor : Subsystem
  body sensor1 : Subsystem
  body sensor2 : Subsystem
  extension torque {,1..3} (4 alike) : Gain  Gain=-1
  tag scope: LBallCnt=global, LHeelCnt=global, LKneeState=global, LdxThigh=global, Lphi12dphi12=global, Lphi23dphi23=global, Lphi34dphi34=global, RBallCnt=global, RHeelCnt=global, RKneeState=global, RdxThigh=global, Rphi12dphi12=global, Rphi23dphi23=global, Rphi34dphi34=global, dxyzHAT=global, dxyzLHip=global, dxyzRHip=global, xyzHAT=global, xyzLHip=global, xyzRHip=global
  wires:
  R Knee Pos Sensor/1 -> Mux4/1
  Left Hip Actuator2/1 -> Mux2/2
  Right Force Plate/2(COP) -> Terminator2/1
  Sum3/1 -> Mux5/1
  Left Ball Contact/1(LHeelCnt) -> L Ball Skin Load Sensor/1
  Left Hip Actuator3/1 -> Mux3/2
  Left Force Plate/1(GRFs) -> Demux1/1
  R Knee Vel Sensor/1 -> Mux4/2
  R Thigh Displacement  Sensor/1 -> [RdxThigh]
  Left Thigh Sensor Sheet/1(dx) -> L Thigh Displacement  Sensor/1
  Left Hip Actuator4/1 -> Mux5/2
  Sum/1 -> Mux/1
  extension torque 2/1 -> R Hip Actuator/1
  body sensor1/2(v [m/s x3]) -> [dxyzLHip]
  Right Ball Contact/1(LHeelCnt) -> R Ball Skin Load Sensor/1
  L Knee Joint Sensor/1 -> [LKneeState]
  Right Force Plate/1(GRFs) -> Demux2/1
  Right Ball Contact/2(GRF [N N]) -> Right Force Plate/1("GRF_Ball [N N] ")
  L Ball Skin Load Sensor/1 -> [LBallCnt]
  L Thigh Displacement  Sensor/1 -> [LdxThigh]
  body sensor2/1(p [m x3]) -> [xyzRHip]
  [LM23] -> L Knee Actuator/1
  [LStance] -> Left Force Plate/Enable
  L Hip Pos Sensor/1 -> Sum/1
  Sum2/1 -> Mux3/1
  Right Heel Contact/1(LHeelCnt) -> R Heel Skin Load Sensor/1
  Mux1/1 -> [Lphi23dphi23], L Knee Joint Sensor/1
  L Knee Vel Sensor/1 -> Mux1/2
  Constant3/1 -> Sum3/2
  Constant/1 -> Sum/2
  [RM12] -> extension torque 3/1
  Right Thigh Sensor Sheet/1(dx) -> R Thigh Displacement  Sensor/1
  L Hip Vel Sensor/1 -> Left Hip Actuator1/1
  L Knee Pos Sensor/1 -> Mux1/1
  body sensor/2(v [m/s x3]) -> [dxyzHAT]
  "extension torque "/1 -> L Hip Actuator/1
  Mux4/1 -> R Knee Joint Sensor/1, [Rphi23dphi23]
  [RM34] -> extension torque 2/1
  body sensor1/1(p [m x3]) -> [xyzLHip]
  body sensor/1(p [m x3]) -> [xyzHAT]
  Mux2/1 -> [Lphi12dphi12]
  R Heel Skin Load Sensor/1 -> [RHeelCnt]
  Left Hip Actuator1/1 -> Mux/2
  L Ankle Pos Sensor/1 -> Sum1/1
  Right Heel Contact/2(GRF [N N]) -> Right Force Plate/2(GRF_Heel [N N])
  Constant1/1 -> Sum1/2
  L Ankle Vel Sensor/1 -> Left Hip Actuator2/1
  L Heel Skin Load Sensor/1 -> [LHeelCnt]
  extension torque 1/1 -> L Ankle Actuator/1
  Left Heel Contact/1(LHeelCnt) -> L Heel Skin Load Sensor/1
  Left Force Plate/2(COP) -> Terminator1/1
  Left Heel Contact/2(GRF [N N]) -> Left Force Plate/2(GRF_Heel [N N])
  Left Ball Contact/2(GRF [N N]) -> Left Force Plate/1("GRF_Ball [N N] ")
  Demux1/1 -> L_GRF/1
  Mux/1 -> [Lphi34dphi34]
  Sum1/1 -> Mux2/1
  Constant2/1 -> Sum2/2
  R Ankle Pos Sensor/1 -> Sum3/1
  Demux2/3 -> R_GRF/3
  [LM12] -> extension torque 1/1
  Demux2/1 -> R_GRF/1
  [RStance] -> Right Force Plate/Enable
  Demux1/3 -> L_GRF/3
  Demux2/2 -> R_GRF/2
  R Ball Skin Load Sensor/1 -> [RBallCnt]
  body sensor2/2(v [m/s x3]) -> [dxyzRHip]
  Demux1/2 -> L_GRF/2
  R Ankle Vel Sensor/1 -> Left Hip Actuator4/1
  extension torque 3/1 -> R Ankle Actuator/1
  Mux5/1 -> [Rphi12dphi12]
  R Knee Joint Sensor/1 -> [RKneeState]
  Mux3/1 -> [Rphi34dphi34]
  R Hip Pos Sensor/1 -> Sum2/1
  R Hip Vel Sensor/1 -> Left Hip Actuator3/1
  [RM23] -> R Knee Actuator/1
  [LM34] -> "extension torque "/1
  [vBelt] -> Left Ball Contact/1(vBelt)
  [vBelt] -> Left Heel Contact/1(vBelt)
  [vBelt] -> Right Heel Contact/1(vBelt)
  [vBelt] -> Right Ball Contact/1(vBelt)
  Treadmill Speed Profile/1 -> Belt Speed/1, belt speed in world frame/1
  belt speed in world frame/1 -> [vBelt]
  connections:
  "Planar Floating Joint "/RConn1 -- HAT (floating base)1/LConn1 -- body sensor/LConn1
  "Planar Floating Joint "/LConn1 -- World Frame/RConn1 -- Mechanism Configuration/RConn1 -- Solver Configuration/RConn1
  Left Hip Joint/LConn1 -- HAT (floating base)1/RConn1 -- body sensor1/LConn1
  Right Hip Joint/LConn1 -- HAT (floating base)1/RConn2 -- body sensor2/LConn1
  Right Foot/LConn1 -- Right Ankle Joint/RConn1
  Right Thigh Sensor Sheet/RConn1 -- Right Thigh Low/LConn1
  Right Shank/RConn1 -- Right Ankle Joint/LConn1
  L Knee Vel Sensor/LConn1 -- Left Knee Joint/RConn3
  Left Knee Joint/RConn2 -- L Knee Pos Sensor/LConn1
  Right Knee Joint/RConn2 -- R Knee Pos Sensor/LConn1
  Right Ball Contact/LConn1 -- Right Foot/RConn1
  Left Thigh Low/RConn1 -- Left Knee Joint/LConn1
  Right Thigh Low/RConn1 -- Right Knee Joint/LConn1
  L Hip Vel Sensor/LConn1 -- Left Hip Joint/RConn3
  Left Thigh High/LConn1 -- Left Hip Joint/RConn1
  R Hip Actuator/RConn1 -- Right Hip Joint/LConn2
  Left Ankle Joint/RConn2 -- L Ankle Pos Sensor/LConn1
  L Ankle Actuator/RConn1 -- Left Ankle Joint/LConn2
  Left Hip Joint/RConn2 -- L Hip Pos Sensor/LConn1
  R Knee Vel Sensor/LConn1 -- Right Knee Joint/RConn3
  L Knee Actuator/RConn1 -- Left Knee Joint/LConn2
  L Ankle Vel Sensor/LConn1 -- Left Ankle Joint/RConn3
  Left Thigh Sensor Sheet/RConn1 -- Left Thigh Low/LConn1
  L Hip Actuator/RConn1 -- Left Hip Joint/LConn2
  "Left Shank "/LConn1 -- Left Knee Joint/RConn1
  Right Hip Joint/RConn2 -- R Hip Pos Sensor/LConn1
  R Knee Actuator/RConn1 -- Right Knee Joint/LConn2
  Left Ball Contact/LConn1 -- Left Foot/RConn1
  "Left Shank "/RConn1 -- Left Ankle Joint/LConn1
  Left Thigh Sensor Sheet/LConn1 -- Left Thigh High/RConn1
  Left Foot/LConn1 -- Left Ankle Joint/RConn1
  R Ankle Vel Sensor/LConn1 -- Right Ankle Joint/RConn3
  Left Heel Contact/LConn1 -- Left Foot/LConn2
  R Hip Vel Sensor/LConn1 -- Right Hip Joint/RConn3
  Right Heel Contact/LConn1 -- Right Foot/LConn2
  Right Shank/LConn1 -- Right Knee Joint/RConn1
  R Ankle Actuator/RConn1 -- Right Ankle Joint/LConn2
  Right Ankle Joint/RConn2 -- R Ankle Pos Sensor/LConn1
  Right Thigh High/LConn1 -- Right Hip Joint/RConn1
  Right Thigh High/RConn1 -- Right Thigh Sensor Sheet/LConn1

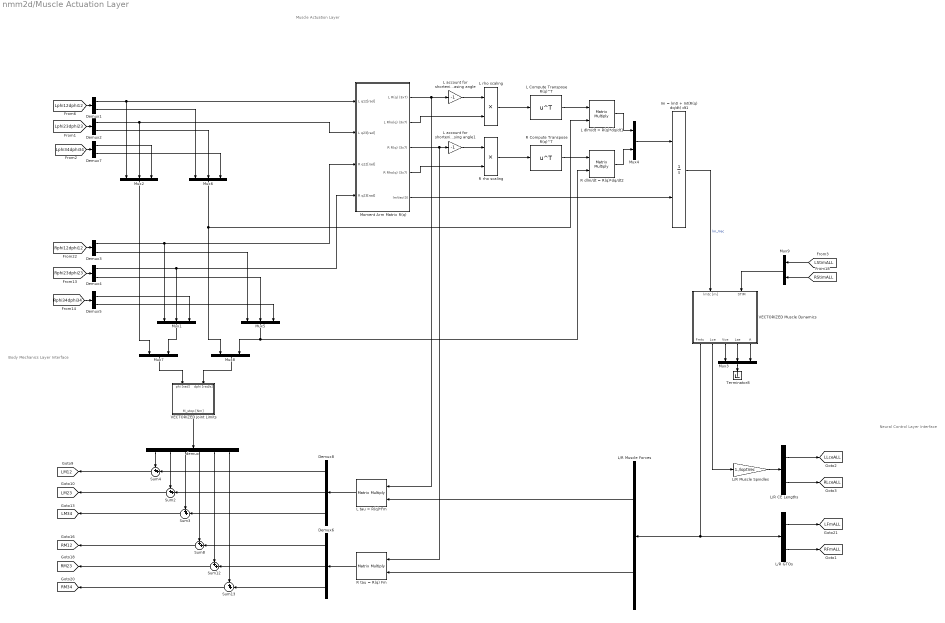
== system nmm2d/Muscle Actuation Layer ==
  note: Muscle Actuation Layer
  note: Neural Control Layer
      | Interface
  note: Body Mechanics Layer
      | Interface
  Demux{1..5,7} (6 alike) : Demux  Outputs=2
  Demux6 : Demux  Outputs=3
  Demux8 : Demux  Outputs=3
  Im = lm0 + Int(R(q) dq/dt) dt1 : Integrator  InitialConditionSource=external
  L rho scaling : Product
  L Compute Transpose R(q)^T : Math  Operator=transpose  SignedPower=on
  L account for shortening/extension of extensors/flexors with increasing angle : Gain  Gain=-1
  L account for shortening/extension of extensors/flexors with increasing angle1 : Gain  Gain=-1
  L dlm/dt = R(q)*dq/dt1 : Product  Multiplication=Matrix(*)
  L tau = R(q)*Fm : Product  Multiplication=Matrix(*)
  L/R Muscle Spindles : Gain  Gain=1./loptVec
  L/R CE Lengths : Demux  Outputs=2
  L/R GTOs : Demux  Outputs=2
  L/R Muscle Forces : Demux  Outputs=2
  Moment Arm Matrix R(q) : Subsystem
  Mux{1..3,5..6} (5 alike) : Mux  Inputs=3
  Mux{4,7..9} (4 alike) : Mux  Inputs=2
  R rho scaling : Product
  R Compute Transpose R(q)^T : Math  Operator=transpose  SignedPower=on
  R dlm/dt = R(q)*dq/dt2 : Product  Multiplication=Matrix(*)
  R tau = R(q) Fm : Product  Multiplication=Matrix(*)
  Sum{2..4,8,12..13} (6 alike) : Sum  Inputs=++|
  Terminator8 : Terminator
  VECTORIZED Muscle Dynamics : Subsystem
  VECTORIZED Joint Limits : Subsystem
  demux : Demux  Outputs=6
  tag scope: LFmALL=global, LLceALL=global, LM12=global, LM23=global, LM34=global, RFmALL=global, RLceALL=global, RM12=global, RM23=global, RM34=global
  wires:
  Demux3/1 -> Mux1/1, Moment Arm Matrix R(q)/3(R q12[rad])
  Demux3/2 -> Mux5/1
  Demux4/2 -> Mux5/2
  [Rphi12dphi12] -> Demux3/1
  [Rphi23dphi23] -> Demux4/1
  [Rphi34dphi34] -> Demux5/1
  Demux5/2 -> Mux5/3
  Demux4/1 -> Mux1/2, Moment Arm Matrix R(q)/4(R q23[rad])
  Sum8/1 -> [RM12]
  Sum12/1 -> [RM23]
  Sum13/1 -> [RM34]
  Demux8/3 -> Sum3/2
  Sum3/1 -> [LM34]
  Demux8/2 -> Sum2/2
  Sum2/1 -> [LM23]
  Demux8/1 -> Sum4/2
  Sum4/1 -> [LM12]
  VECTORIZED Muscle Dynamics/2(Lce) -> L/R Muscle Spindles/1
  VECTORIZED Muscle Dynamics/5(A) -> Mux3/3
  VECTORIZED Muscle Dynamics/4(Lse) -> Mux3/2
  VECTORIZED Muscle Dynamics/3(Vce) -> Mux3/1
  Mux3/1 -> Terminator8/1
  [LStimALL] -> Mux9/1
  L account for shortening/extension of extensors/flexors with increasing angle/1 -> L rho scaling/1
  Moment Arm Matrix R(q)/1(L R(q) (3x7)) -> L tau = R(q)*Fm/1, L account for shortening/extension of extensors/flexors with increasing angle/1
  L tau = R(q)*Fm/1 -> Demux8/1
  Demux2/1 -> Moment Arm Matrix R(q)/2(L q23[rad]), Mux2/2
  L Compute Transpose R(q)^T/1 -> L dlm/dt = R(q)*dq/dt1/1
  Moment Arm Matrix R(q)/2(L Rho(q) (3x7)) -> L rho scaling/2
  L rho scaling/1 -> L Compute Transpose R(q)^T/1
  Im = lm0 + Int(R(q) dq/dt) dt1/1 -> VECTORIZED Muscle Dynamics/1(lmtc [m])  "lm_Vec"
  Moment Arm Matrix R(q)/5(lmVec(0)) -> Im = lm0 + Int(R(q) dq/dt) dt1/2
  Demux7/2 -> Mux6/3
  [Lphi34dphi34] -> Demux7/1
  [Lphi23dphi23] -> Demux2/1
  [Lphi12dphi12] -> Demux1/1
  Demux2/2 -> Mux6/2
  Demux1/2 -> Mux6/1
  Demux1/1 -> Moment Arm Matrix R(q)/1(L q12[rad]), Mux2/1
  [RStimALL] -> Mux9/2
  Mux9/1 -> VECTORIZED Muscle Dynamics/2(STIM)
  Mux6/1 -> L dlm/dt = R(q)*dq/dt1/2, Mux8/1
  Demux6/2 -> Sum12/2
  Demux6/1 -> Sum8/2
  Demux6/3 -> Sum13/2
  R tau = R(q) Fm/1 -> Demux6/1
  L account for shortening/extension of extensors/flexors with increasing angle1/1 -> R rho scaling/1
  R rho scaling/1 -> R Compute Transpose R(q)^T/1
  R Compute Transpose R(q)^T/1 -> R dlm/dt = R(q)*dq/dt2/1
  Mux5/1 -> Mux8/2, R dlm/dt = R(q)*dq/dt2/2
  L dlm/dt = R(q)*dq/dt1/1 -> Mux4/1
  R dlm/dt = R(q)*dq/dt2/1 -> Mux4/2
  Mux4/1 -> Im = lm0 + Int(R(q) dq/dt) dt1/1
  L/R Muscle Forces/1 -> L tau = R(q)*Fm/2
  Moment Arm Matrix R(q)/4(R Rho(q) (3x7)) -> R rho scaling/2
  Moment Arm Matrix R(q)/3(R R(q) (3x7)) -> R tau = R(q) Fm/1, L account for shortening/extension of extensors/flexors with increasing angle1/1
  L/R CE Lengths/1 -> [LLceALL]
  L/R CE Lengths/2 -> [RLceALL]
  L/R Muscle Forces/2 -> R tau = R(q) Fm/2
  L/R GTOs/1 -> [LFmALL]
  L/R GTOs/2 -> [RFmALL]
  L/R Muscle Spindles/1 -> L/R CE Lengths/1
  demux/1 -> Sum4/1
  demux/2 -> Sum2/1
  demux/3 -> Sum3/1
  VECTORIZED Joint Limits/1(M_stop [Nm]) -> demux/1
  demux/4 -> Sum8/1
  demux/5 -> Sum12/1
  demux/6 -> Sum13/1
  Demux7/1 -> Mux2/3
  Demux5/1 -> Mux1/3
  Mux1/1 -> Mux7/2
  Mux2/1 -> Mux7/1
  Mux7/1 -> VECTORIZED Joint Limits/1(phi [rad])
  Mux8/1 -> VECTORIZED Joint Limits/2(dphi [rad/s])
  VECTORIZED Muscle Dynamics/1(Fmtc) -> L/R GTOs/1, L/R Muscle Forces/1
